simulink model "GalacticSoupFunctional"  (R2026a)
settings: Solver=VariableStepAuto
settings Model: DataDictionary=FunctionalInterfaces.sldd  Creator=sarah  LastModifiedBy=sarah

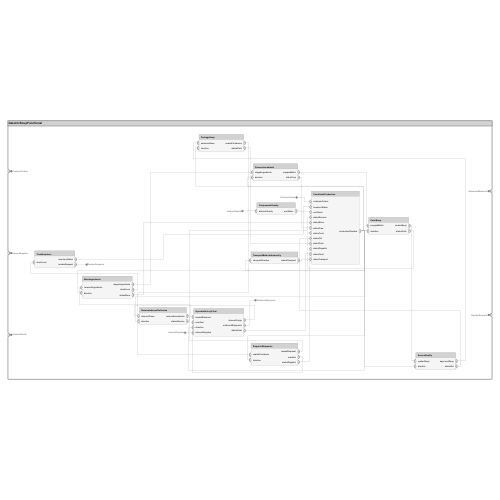
[thumbnail: Simulink's stored preview of the top-level diagram]
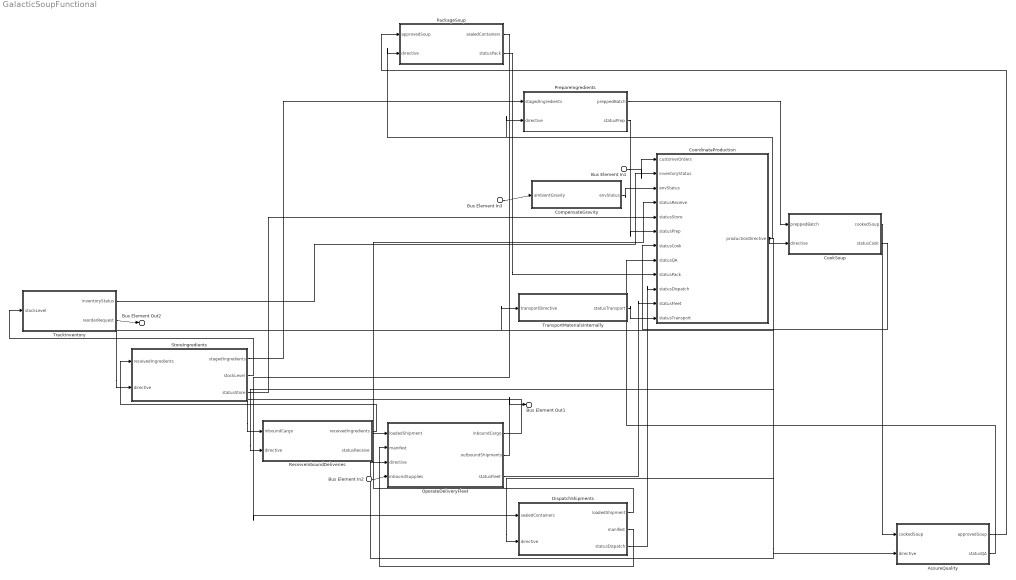
== system GalacticSoupFunctional ==
  Bus Element In1 : Inport  PortName=CustomerOrders
  Bus Element In2 : Inport  Port=2  PortName=InboundSupplies
  Bus Element In3 : Inport  Port=3  PortName=AmbientGravity
  AssureQuality : Subsystem
      settings: PortSchema="{\"entries\":[{\"content\":{\"headerSize\":26,\"margin\":15,\"minimumSpacing\":25,\"sides\":[{\"content\":{\"connectorIds\":[\"In1\",\"In2\"]},\"type\":\"ConnectorPlacement.EquallySpacedRectSide\",\"uuid\":\"f830f98a-8e8b-4468-adf4-d6eab644987f\"},{\"content\":{\"connectorIds\":[\"Out1\",\"Out2\"],\"side\":\"RIGHT\"},\"type\":\"ConnectorPlacement.EquallySpacedRectSide\",\"uuid\":\"7e0d0116-b3ba-4668-b638-30d0f54ba087\"},{\"content\":{\"side\":\"TOP\"},\"type\":\"ConnectorPlacement.EquallySpacedRectSide\",\"uuid\":\"7b4146d3-46d2-45ca-8c34-b106f0d8cedd\"}]},\"type\":\"ConnectorPlacement.EquallySpacedConnector\",\"uuid\":\"3d911b2d-a78f-42ea-b869-5e09982d9f54\"}],\"packageUris\":[\"http://schema.mathworks.com/mf0/Connector/R2020b\"],\"version\":\"1.0\"}"
  CompensateGravity : Subsystem
      settings: PortSchema="{\"entries\":[{\"content\":{\"headerSize\":26,\"margin\":15,\"minimumSpacing\":25,\"sides\":[{\"content\":{\"connectorIds\":[\"In1\"]},\"type\":\"ConnectorPlacement.EquallySpacedRectSide\",\"uuid\":\"f830f98a-8e8b-4468-adf4-d6eab644987f\"},{\"content\":{\"connectorIds\":[\"Out1\"],\"side\":\"RIGHT\"},\"type\":\"ConnectorPlacement.EquallySpacedRectSide\",\"uuid\":\"7e0d0116-b3ba-4668-b638-30d0f54ba087\"},{\"content\":{\"side\":\"TOP\"},\"type\":\"ConnectorPlacement.EquallySpacedRectSide\",\"uuid\":\"7b4146d3-46d2-45ca-8c34-b106f0d8cedd\"}]},\"type\":\"ConnectorPlacement.EquallySpacedConnector\",\"uuid\":\"3d911b2d-a78f-42ea-b869-5e09982d9f54\"}],\"packageUris\":[\"http://schema.mathworks.com/mf0/Connector/R2020b\"],\"version\":\"1.0\"}"
  CookSoup : Subsystem
      settings: PortSchema="{\"entries\":[{\"content\":{\"headerSize\":26,\"margin\":15,\"minimumSpacing\":25,\"sides\":[{\"content\":{\"connectorIds\":[\"In1\",\"In2\"]},\"type\":\"ConnectorPlacement.EquallySpacedRectSide\",\"uuid\":\"f830f98a-8e8b-4468-adf4-d6eab644987f\"},{\"content\":{\"connectorIds\":[\"Out1\",\"Out2\"],\"side\":\"RIGHT\"},\"type\":\"ConnectorPlacement.EquallySpacedRectSide\",\"uuid\":\"7e0d0116-b3ba-4668-b638-30d0f54ba087\"},{\"content\":{\"side\":\"TOP\"},\"type\":\"ConnectorPlacement.EquallySpacedRectSide\",\"uuid\":\"7b4146d3-46d2-45ca-8c34-b106f0d8cedd\"}]},\"type\":\"ConnectorPlacement.EquallySpacedConnector\",\"uuid\":\"3d911b2d-a78f-42ea-b869-5e09982d9f54\"}],\"packageUris\":[\"http://schema.mathworks.com/mf0/Connector/R2020b\"],\"version\":\"1.0\"}"
  CoordinateProduction : Subsystem
      settings: PortSchema="{\"entries\":[{\"content\":{\"headerSize\":26,\"margin\":15,\"minimumSpacing\":25,\"sides\":[{\"content\":{\"connectorIds\":[\"In1\",\"In2\",\"In3\",\"In4\",\"In5\",\"In6\",\"In7\",\"In8\",\"In9\",\"In10\",\"In11\",\"In12\"]},\"type\":\"ConnectorPlacement.EquallySpacedRectSide\",\"uuid\":\"f830f98a-8e8b-4468-adf4-d6eab644987f\"},{\"content\":{\"connectorIds\":[\"Out1\"],\"side\":\"RIGHT\"},\"type\":\"ConnectorPlacement.EquallySpacedRectSide\",\"uuid\":\"7e0d0116-b3ba-4668-b638-30d0f54ba087\"},{\"content\":{\"side\":\"TOP\"},\"type\":\"ConnectorPlacement.EquallySpacedRectSide\",\"uuid\":\"7b4146d3-46d2-45ca-8c34-b106f0d8cedd\"}]},\"type\":\"ConnectorPlacement.EquallySpacedConnector\",\"uuid\":\"3d911b2d-a78f-42ea-b869-5e09982d9f54\"}],\"packageUris\":[\"http://schema.mathworks.com/mf0/Connector/R2020b\"],\"version\":\"1.0\"}"
  DispatchShipments : Subsystem
      settings: PortSchema="{\"entries\":[{\"content\":{\"headerSize\":26,\"margin\":15,\"minimumSpacing\":25,\"sides\":[{\"content\":{\"connectorIds\":[\"In1\",\"In2\"]},\"type\":\"ConnectorPlacement.EquallySpacedRectSide\",\"uuid\":\"f830f98a-8e8b-4468-adf4-d6eab644987f\"},{\"content\":{\"connectorIds\":[\"Out1\",\"Out2\",\"Out3\"],\"side\":\"RIGHT\"},\"type\":\"ConnectorPlacement.EquallySpacedRectSide\",\"uuid\":\"7e0d0116-b3ba-4668-b638-30d0f54ba087\"},{\"content\":{\"side\":\"TOP\"},\"type\":\"ConnectorPlacement.EquallySpacedRectSide\",\"uuid\":\"7b4146d3-46d2-45ca-8c34-b106f0d8cedd\"}]},\"type\":\"ConnectorPlacement.EquallySpacedConnector\",\"uuid\":\"3d911b2d-a78f-42ea-b869-5e09982d9f54\"}],\"packageUris\":[\"http://schema.mathworks.com/mf0/Connector/R2020b\"],\"version\":\"1.0\"}"
  OperateDeliveryFleet : Subsystem
      settings: PortSchema="{\"entries\":[{\"content\":{\"headerSize\":26,\"margin\":15,\"minimumSpacing\":25,\"sides\":[{\"content\":{\"connectorIds\":[\"In1\",\"In2\",\"In3\",\"In4\"]},\"type\":\"ConnectorPlacement.EquallySpacedRectSide\",\"uuid\":\"f830f98a-8e8b-4468-adf4-d6eab644987f\"},{\"content\":{\"connectorIds\":[\"Out1\",\"Out2\",\"Out3\"],\"side\":\"RIGHT\"},\"type\":\"ConnectorPlacement.EquallySpacedRectSide\",\"uuid\":\"7e0d0116-b3ba-4668-b638-30d0f54ba087\"},{\"content\":{\"side\":\"TOP\"},\"type\":\"ConnectorPlacement.EquallySpacedRectSide\",\"uuid\":\"7b4146d3-46d2-45ca-8c34-b106f0d8cedd\"}]},\"type\":\"ConnectorPlacement.EquallySpacedConnector\",\"uuid\":\"3d911b2d-a78f-42ea-b869-5e09982d9f54\"}],\"packageUris\":[\"http://schema.mathworks.com/mf0/Connector/R2020b\"],\"version\":\"1.0\"}"
  PackageSoup : Subsystem
      settings: PortSchema="{\"entries\":[{\"content\":{\"headerSize\":26,\"margin\":15,\"minimumSpacing\":25,\"sides\":[{\"content\":{\"connectorIds\":[\"In1\",\"In2\"]},\"type\":\"ConnectorPlacement.EquallySpacedRectSide\",\"uuid\":\"f830f98a-8e8b-4468-adf4-d6eab644987f\"},{\"content\":{\"connectorIds\":[\"Out1\",\"Out2\"],\"side\":\"RIGHT\"},\"type\":\"ConnectorPlacement.EquallySpacedRectSide\",\"uuid\":\"7e0d0116-b3ba-4668-b638-30d0f54ba087\"},{\"content\":{\"side\":\"TOP\"},\"type\":\"ConnectorPlacement.EquallySpacedRectSide\",\"uuid\":\"7b4146d3-46d2-45ca-8c34-b106f0d8cedd\"}]},\"type\":\"ConnectorPlacement.EquallySpacedConnector\",\"uuid\":\"3d911b2d-a78f-42ea-b869-5e09982d9f54\"}],\"packageUris\":[\"http://schema.mathworks.com/mf0/Connector/R2020b\"],\"version\":\"1.0\"}"
  PrepareIngredients : Subsystem
      settings: PortSchema="{\"entries\":[{\"content\":{\"headerSize\":26,\"margin\":15,\"minimumSpacing\":25,\"sides\":[{\"content\":{\"connectorIds\":[\"In1\",\"In2\"]},\"type\":\"ConnectorPlacement.EquallySpacedRectSide\",\"uuid\":\"f830f98a-8e8b-4468-adf4-d6eab644987f\"},{\"content\":{\"connectorIds\":[\"Out1\",\"Out2\"],\"side\":\"RIGHT\"},\"type\":\"ConnectorPlacement.EquallySpacedRectSide\",\"uuid\":\"7e0d0116-b3ba-4668-b638-30d0f54ba087\"},{\"content\":{\"side\":\"TOP\"},\"type\":\"ConnectorPlacement.EquallySpacedRectSide\",\"uuid\":\"7b4146d3-46d2-45ca-8c34-b106f0d8cedd\"}]},\"type\":\"ConnectorPlacement.EquallySpacedConnector\",\"uuid\":\"3d911b2d-a78f-42ea-b869-5e09982d9f54\"}],\"packageUris\":[\"http://schema.mathworks.com/mf0/Connector/R2020b\"],\"version\":\"1.0\"}"
  ReceiveInboundDeliveries : Subsystem
      settings: PortSchema="{\"entries\":[{\"content\":{\"headerSize\":26,\"margin\":15,\"minimumSpacing\":25,\"sides\":[{\"content\":{\"connectorIds\":[\"In1\",\"In2\"]},\"type\":\"ConnectorPlacement.EquallySpacedRectSide\",\"uuid\":\"f830f98a-8e8b-4468-adf4-d6eab644987f\"},{\"content\":{\"connectorIds\":[\"Out1\",\"Out2\"],\"side\":\"RIGHT\"},\"type\":\"ConnectorPlacement.EquallySpacedRectSide\",\"uuid\":\"7e0d0116-b3ba-4668-b638-30d0f54ba087\"},{\"content\":{\"side\":\"TOP\"},\"type\":\"ConnectorPlacement.EquallySpacedRectSide\",\"uuid\":\"7b4146d3-46d2-45ca-8c34-b106f0d8cedd\"}]},\"type\":\"ConnectorPlacement.EquallySpacedConnector\",\"uuid\":\"3d911b2d-a78f-42ea-b869-5e09982d9f54\"}],\"packageUris\":[\"http://schema.mathworks.com/mf0/Connector/R2020b\"],\"version\":\"1.0\"}"
  StoreIngredients : Subsystem
      settings: PortSchema="{\"entries\":[{\"content\":{\"headerSize\":26,\"margin\":15,\"minimumSpacing\":25,\"sides\":[{\"content\":{\"connectorIds\":[\"In1\",\"In2\"]},\"type\":\"ConnectorPlacement.EquallySpacedRectSide\",\"uuid\":\"f830f98a-8e8b-4468-adf4-d6eab644987f\"},{\"content\":{\"connectorIds\":[\"Out1\",\"Out2\",\"Out3\"],\"side\":\"RIGHT\"},\"type\":\"ConnectorPlacement.EquallySpacedRectSide\",\"uuid\":\"7e0d0116-b3ba-4668-b638-30d0f54ba087\"},{\"content\":{\"side\":\"TOP\"},\"type\":\"ConnectorPlacement.EquallySpacedRectSide\",\"uuid\":\"7b4146d3-46d2-45ca-8c34-b106f0d8cedd\"}]},\"type\":\"ConnectorPlacement.EquallySpacedConnector\",\"uuid\":\"3d911b2d-a78f-42ea-b869-5e09982d9f54\"}],\"packageUris\":[\"http://schema.mathworks.com/mf0/Connector/R2020b\"],\"version\":\"1.0\"}"
  TrackInventory : Subsystem
      settings: PortSchema="{\"entries\":[{\"content\":{\"headerSize\":26,\"margin\":15,\"minimumSpacing\":25,\"sides\":[{\"content\":{\"connectorIds\":[\"In1\"]},\"type\":\"ConnectorPlacement.EquallySpacedRectSide\",\"uuid\":\"f830f98a-8e8b-4468-adf4-d6eab644987f\"},{\"content\":{\"connectorIds\":[\"Out1\",\"Out2\"],\"side\":\"RIGHT\"},\"type\":\"ConnectorPlacement.EquallySpacedRectSide\",\"uuid\":\"7e0d0116-b3ba-4668-b638-30d0f54ba087\"},{\"content\":{\"side\":\"TOP\"},\"type\":\"ConnectorPlacement.EquallySpacedRectSide\",\"uuid\":\"7b4146d3-46d2-45ca-8c34-b106f0d8cedd\"}]},\"type\":\"ConnectorPlacement.EquallySpacedConnector\",\"uuid\":\"3d911b2d-a78f-42ea-b869-5e09982d9f54\"}],\"packageUris\":[\"http://schema.mathworks.com/mf0/Connector/R2020b\"],\"version\":\"1.0\"}"
  TransportMaterialsInternally : Subsystem
      settings: PortSchema="{\"entries\":[{\"content\":{\"headerSize\":26,\"margin\":15,\"minimumSpacing\":25,\"sides\":[{\"content\":{\"connectorIds\":[\"In1\"]},\"type\":\"ConnectorPlacement.EquallySpacedRectSide\",\"uuid\":\"f830f98a-8e8b-4468-adf4-d6eab644987f\"},{\"content\":{\"connectorIds\":[\"Out1\"],\"side\":\"RIGHT\"},\"type\":\"ConnectorPlacement.EquallySpacedRectSide\",\"uuid\":\"7e0d0116-b3ba-4668-b638-30d0f54ba087\"},{\"content\":{\"side\":\"TOP\"},\"type\":\"ConnectorPlacement.EquallySpacedRectSide\",\"uuid\":\"7b4146d3-46d2-45ca-8c34-b106f0d8cedd\"}]},\"type\":\"ConnectorPlacement.EquallySpacedConnector\",\"uuid\":\"3d911b2d-a78f-42ea-b869-5e09982d9f54\"}],\"packageUris\":[\"http://schema.mathworks.com/mf0/Connector/R2020b\"],\"version\":\"1.0\"}"
  Bus Element Out1 : Outport  PortName=OutboundShipments
  Bus Element Out2 : Outport  Port=2  PortName=ReorderRequests
  wires:
  ReceiveInboundDeliveries/1(receivedIngredients) -> StoreIngredients/1(receivedIngredients)
  TrackInventory/1(inventoryStatus) -> CoordinateProduction/2(inventoryStatus)
  ReceiveInboundDeliveries/2(statusReceive) -> CoordinateProduction/4(statusReceive)
  StoreIngredients/1(stagedIngredients) -> PrepareIngredients/1(stagedIngredients)
  TrackInventory/2(reorderRequest) -> Bus Element Out2/1
  StoreIngredients/2(stockLevel) -> TrackInventory/1(stockLevel)
  StoreIngredients/3(statusStore) -> CoordinateProduction/5(statusStore)
  Bus Element In2/1 -> OperateDeliveryFleet/4(inboundSupplies)
  TransportMaterialsInternally/1(statusTransport) -> CoordinateProduction/12(statusTransport)
  PackageSoup/1(sealedContainers) -> DispatchShipments/1(sealedContainers)
  PackageSoup/2(statusPack) -> CoordinateProduction/9(statusPack)
  Bus Element In3/1 -> CompensateGravity/1(ambientGravity)
  DispatchShipments/3(statusDispatch) -> CoordinateProduction/10(statusDispatch)
  OperateDeliveryFleet/1(inboundCargo) -> ReceiveInboundDeliveries/1(inboundCargo)
  PrepareIngredients/1(preppedBatch) -> CookSoup/1(preppedBatch)
  OperateDeliveryFleet/2(outboundShipments) -> Bus Element Out1/1
  PrepareIngredients/2(statusPrep) -> CoordinateProduction/6(statusPrep)
  OperateDeliveryFleet/3(statusFleet) -> CoordinateProduction/11(statusFleet)
  Bus Element In1/1 -> CoordinateProduction/1(customerOrders)
  CompensateGravity/1(envStatus) -> CoordinateProduction/3(envStatus)
  DispatchShipments/1(loadedShipment) -> OperateDeliveryFleet/1(loadedShipment)
  DispatchShipments/2(manifest) -> OperateDeliveryFleet/2(manifest)
  CoordinateProduction/1(productionDirective) -> OperateDeliveryFleet/3(directive), PackageSoup/2(directive), TransportMaterialsInternally/1(transportDirective), StoreIngredients/2(directive), PrepareIngredients/2(directive), ReceiveInboundDeliveries/2(directive), AssureQuality/2(directive), DispatchShipments/2(directive), CookSoup/2(directive)
  CookSoup/1(cookedSoup) -> AssureQuality/1(cookedSoup)
  CookSoup/2(statusCook) -> CoordinateProduction/7(statusCook)
  AssureQuality/1(approvedSoup) -> PackageSoup/1(approvedSoup)
  AssureQuality/2(statusQA) -> CoordinateProduction/8(statusQA)

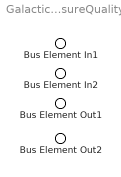
== system GalacticSoupFunctional/AssureQuality ==
  Bus Element In1 : Inport  PortName=cookedSoup
  Bus Element In2 : Inport  Port=2  PortName=directive
  Bus Element Out1 : Outport  PortName=approvedSoup
  Bus Element Out2 : Outport  Port=2  PortName=statusQA

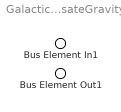
== system GalacticSoupFunctional/CompensateGravity ==
  Bus Element In1 : Inport  PortName=ambientGravity
  Bus Element Out1 : Outport  PortName=envStatus

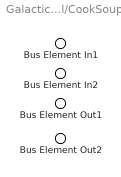
== system GalacticSoupFunctional/CookSoup ==
  Bus Element In1 : Inport  PortName=preppedBatch
  Bus Element In2 : Inport  Port=2  PortName=directive
  Bus Element Out1 : Outport  PortName=cookedSoup
  Bus Element Out2 : Outport  Port=2  PortName=statusCook

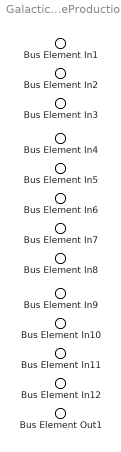
== system GalacticSoupFunctional/CoordinateProduction ==
  Bus Element In1 : Inport  PortName=customerOrders
  Bus Element In2 : Inport  Port=2  PortName=inventoryStatus
  Bus Element In3 : Inport  Port=3  PortName=envStatus
  Bus Element In4 : Inport  Port=4  PortName=statusReceive
  Bus Element In5 : Inport  Port=5  PortName=statusStore
  Bus Element In6 : Inport  Port=6  PortName=statusPrep
  Bus Element In7 : Inport  Port=7  PortName=statusCook
  Bus Element In8 : Inport  Port=8  PortName=statusQA
  Bus Element In9 : Inport  Port=9  PortName=statusPack
  Bus Element In10 : Inport  Port=10  PortName=statusDispatch
  Bus Element In11 : Inport  Port=11  PortName=statusFleet
  Bus Element In12 : Inport  Port=12  PortName=statusTransport
  Bus Element Out1 : Outport  PortName=productionDirective

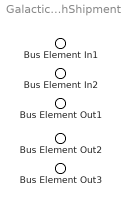
== system GalacticSoupFunctional/DispatchShipments ==
  Bus Element In1 : Inport  PortName=sealedContainers
  Bus Element In2 : Inport  Port=2  PortName=directive
  Bus Element Out1 : Outport  PortName=loadedShipment
  Bus Element Out2 : Outport  Port=2  PortName=manifest
  Bus Element Out3 : Outport  Port=3  PortName=statusDispatch

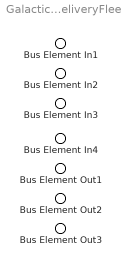
== system GalacticSoupFunctional/OperateDeliveryFleet ==
  Bus Element In1 : Inport  PortName=loadedShipment
  Bus Element In2 : Inport  Port=2  PortName=manifest
  Bus Element In3 : Inport  Port=3  PortName=directive
  Bus Element In4 : Inport  Port=4  PortName=inboundSupplies
  Bus Element Out1 : Outport  PortName=inboundCargo
  Bus Element Out2 : Outport  Port=2  PortName=outboundShipments
  Bus Element Out3 : Outport  Port=3  PortName=statusFleet

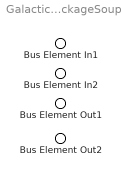
== system GalacticSoupFunctional/PackageSoup ==
  Bus Element In1 : Inport  PortName=approvedSoup
  Bus Element In2 : Inport  Port=2  PortName=directive
  Bus Element Out1 : Outport  PortName=sealedContainers
  Bus Element Out2 : Outport  Port=2  PortName=statusPack

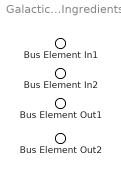
== system GalacticSoupFunctional/PrepareIngredients ==
  Bus Element In1 : Inport  PortName=stagedIngredients
  Bus Element In2 : Inport  Port=2  PortName=directive
  Bus Element Out1 : Outport  PortName=preppedBatch
  Bus Element Out2 : Outport  Port=2  PortName=statusPrep

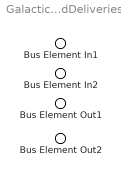
== system GalacticSoupFunctional/ReceiveInboundDeliveries ==
  Bus Element In1 : Inport  PortName=inboundCargo
  Bus Element In2 : Inport  Port=2  PortName=directive
  Bus Element Out1 : Outport  PortName=receivedIngredients
  Bus Element Out2 : Outport  Port=2  PortName=statusReceive

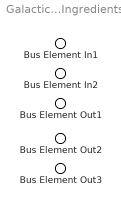
== system GalacticSoupFunctional/StoreIngredients ==
  Bus Element In1 : Inport  PortName=receivedIngredients
  Bus Element In2 : Inport  Port=2  PortName=directive
  Bus Element Out1 : Outport  PortName=stagedIngredients
  Bus Element Out2 : Outport  Port=2  PortName=stockLevel
  Bus Element Out3 : Outport  Port=3  PortName=statusStore

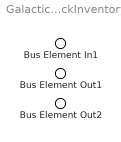
== system GalacticSoupFunctional/TrackInventory ==
  Bus Element In1 : Inport  PortName=stockLevel
  Bus Element Out1 : Outport  PortName=inventoryStatus
  Bus Element Out2 : Outport  Port=2  PortName=reorderRequest

== system GalacticSoupFunctional/TransportMaterialsInternally ==
  Bus Element In1 : Inport  PortName=transportDirective
  Bus Element Out1 : Outport  PortName=statusTransport
